simulink model "fopid"  (R2025b)
settings: Solver=FixedStepAuto  StartTime=0.0  StopTime=10.0  FixedStep=0.001  RelTol=1e-3
libraries: fod x1, slpidlib x1
settings Model: Creator=chen'z'y  LastModifiedBy=chen'z'y

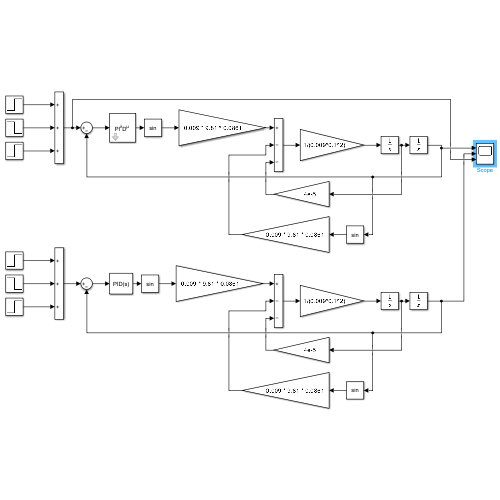
[thumbnail: Simulink's stored preview of the top-level diagram]
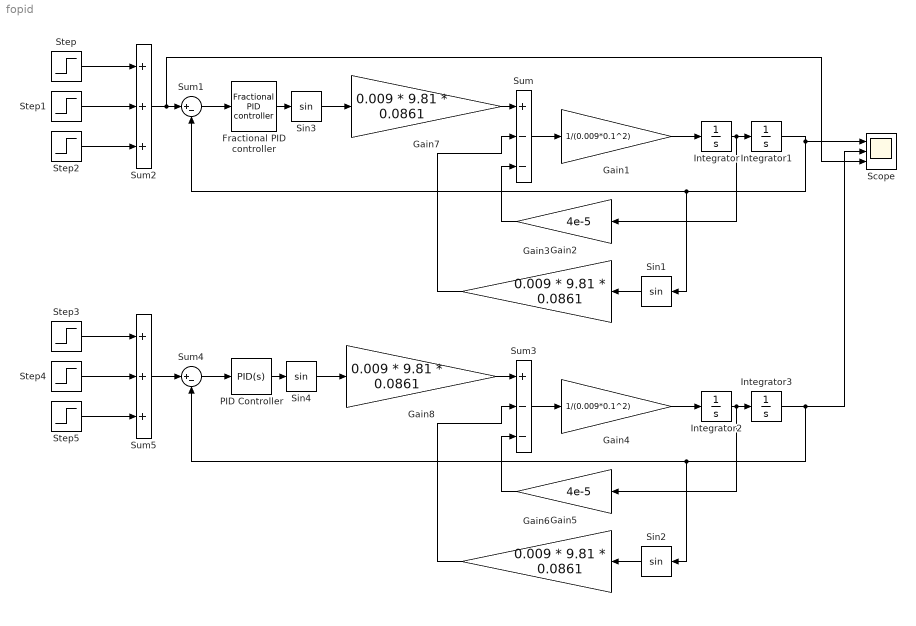
== system fopid ==
  Fractional PID controller : fod/Fractional PID controller  Kp=1  Ki=9.0747  lambda=0.95  Kd=0.3036  mic=0.95  freqRange=[0.01, 1000]  N=5
      settings: SourceProductName=FOMCON Toolbox
  Gain1 : Gain  Gain=1/(0.009*0.1^2)
  Gain2 : Gain  Gain=4e-5
  Gain{3,6..8} (4 alike) : Gain  Gain=0.009 * 9.81 * 0.0861
  Gain4 : Gain  Gain=1/(0.009*0.1^2)
  Gain5 : Gain  Gain=4e-5
  Integrator{,1..3} (4 alike) : Integrator
  PID Controller : slpidlib/PID Controller  Controller=PID  Form=Parallel  TimeDomain=Continuous-time  UseExternalTs=off  SampleTime=-1  IntegratorMethod=Forward Euler  FilterMethod=Forward Euler  ControllerParametersSource=internal  P=1  I=9.0747  UseKiTs=off  D=0.3036  UseExternalDerivativeSource=off  N=100  UseFilter=on  TunerSelectOption=Transfer Function Based (PID Tuner App)  InitialConditionSource=internal  InitialConditionForIntegrator=0  InitialConditionForFilter=0  DifferentiatorICPrevScaledInput=0  ExternalReset=none  TrackingMode=off  Kt=1  LimitOutput=off  SatLimitsSource=internal  UpperSaturationLimit=inf  LowerSaturationLimit=-inf  LinearizeAsGain=on  AntiWindupMode=none  Kb=1  LimitIntegrator=off  UpperIntegratorSaturationLimit=inf  LowerIntegratorSaturationLimit=-inf  POutMin=[]  POutMax=[]  IOutMin=[]  IOutMax=[]  DOutMin=[]  DOutMax=[]  NOutMin=[]  NOutMax=[]  SumOutMin=[]  SumOutMax=[]  SaturationOutMin=[]  SaturationOutMax=[]  PParamMin=[]  PParamMax=[]  IParamMin=[]  IParamMax=[]  DParamMin=[]  DParamMax=[]  NParamMin=[]  NParamMax=[]  KbParamMin=[]  KbParamMax=[]  KtParamMin=[]  KtParamMax=[]  KbOutMin=[]  KbOutMax=[]  KtOutMin=[]  KtOutMax=[]  IntegratorOutMin=[]  IntegratorOutMax=[]  FilterOutMin=[]  FilterOutMax=[]  SumI1OutMin=[]  SumI1OutMax=[]  SumI2OutMin=[]  SumI2OutMax=[]  SumI3OutMin=[]  SumI3OutMax=[]  SumI4OutMin=[]  SumI4OutMax=[]  SumDOutMin=[]  SumDOutMax=[]  DifferentiatorOutMin=[]  DifferentiatorOutMax=[]  FilterDiffOutCoefMin=[]  FilterDiffOutCoefMax=[]  ReciprocalOutMin=[]  ReciprocalOutMax=[]  SumDenOutMin=[]  SumDenOutMax=[]  SumNumOutMin=[]  SumNumOutMax=[]  DivideOutMin=[]  DivideOutMax=[]  UdiffTsProdOutMin=[]  UdiffTsProdOutMax=[]  NTsProdOutMin=[]  NTsProdOutMax=[]  UintegralTsProdOutMin=[]  UintegralTsProdOutMax=[]  UngainTsProdOutMin=[]  UngainTsProdOutMax=[]  ClampingZeroOutDataTypeStr=Inherit: Inherit via back propagation  ClampingZeroOutMin=[]  ClampingZeroOutMax=[]  FilterDenConstantOutDataTypeStr=Inherit: Inherit via back propagation  FilterDenConstantOutMin=[]  FilterDenConstantOutMax=[]  PCopyOutDataTypeStr=Inherit: Inherit via back propagation  PCopyOutMin=[]  PCopyOutMax=[]  NCopyOutDataTypeStr=Inherit: Inherit via back propagation  NCopyOutMin=[]  NCopyOutMax=[]  IntegratorContinuousStateAttributes=''  IntegratorStateMustResolveToSignalObject=off  IntegratorRTWStateStorageClass=Auto  FilterContinuousStateAttributes=''  FilterStateMustResolveToSignalObject=off  FilterRTWStateStorageClass=Auto  ParallelPVariant=InternalParameters  IdealPVariant=Disabled  IVariant=InternalParameters  DVariant=InternalParameters  IntegratorVariant=Continuous  SatVariant=Disabled  AWVariant=Passthrough  PCopyVariant=Disabled  TRVariant=Disabled  FdbkBlocksVariant=Forward  IdealPFdbkVariant=Disabled  SatFdbkVariant=Disabled  DerivativeFilterVariant=ContFilter  NVariant=InternalParameters  NCopyVariant=Disabled  FilterICVariant=InternalICsFilter  IntegratorICVariant=InternalICs  ExternalResetVariant=Disabled  TRSumVariant=Passthrough  SumFdbkVariant=Disabled  SumVariant=Sum_PID  TsampFilterVariant=InternalTs  TsampNgainVariant=Passthrough  TsampIntegralVariant=Disabled_SignalSpec  ExternalSaturationOutDataTypeStr=Inherit: Same as second input  DerivativeSourceVariant=ErrorSignal  PreIntVariant=InternalPreInt
  Scope : Scope  NumInputPorts=3
      settings: ActiveDisplayYMinimum=-0.1114400618964623  ActiveDisplayYMaximum=0.97065217865255393  DataLoggingVariableName=scope_data
  Sin{1..4} (4 alike) : Trigonometry
  Step : Step  Time=0  After=0.6  SampleTime=0
  Step1 : Step  Time=3  After=-0.35  SampleTime=0
  Step2 : Step  Time=7  After=0.5  SampleTime=0
  Step3 : Step  Time=0  After=0.6  SampleTime=0
  Step4 : Step  Time=3  After=-0.35  SampleTime=0
  Step5 : Step  Time=7  After=0.5  SampleTime=0
  Sum : Sum  Inputs=+--
  Sum1 : Sum  Inputs=|+-
  Sum2 : Sum  Inputs=+++
  Sum3 : Sum  Inputs=+--
  Sum4 : Sum  Inputs=|+-
  Sum5 : Sum  Inputs=+++
  wires:
  Sum/1 -> Gain1/1
  Gain1/1 -> Integrator/1
  Integrator/1 -> Gain2/1, Integrator1/1
  Sin1/1 -> Gain3/1
  Gain2/1 -> Sum/3
  Gain3/1 -> Sum/2
  Sum1/1 -> Fractional PID controller/1
  Integrator1/1 -> Scope/1, Sum1/2, Sin1/1
  Sum2/1 -> Scope/3, Sum1/1
  Step2/1 -> Sum2/3
  Step1/1 -> Sum2/2
  Step/1 -> Sum2/1
  Sum5/1 -> Sum4/1
  Gain5/1 -> Sum3/3
  Gain4/1 -> Integrator2/1
  Integrator3/1 -> Scope/2, Sin2/1, Sum4/2
  Sum3/1 -> Gain4/1
  Step5/1 -> Sum5/3
  Sin2/1 -> Gain6/1
  Step3/1 -> Sum5/1
  Gain6/1 -> Sum3/2
  Step4/1 -> Sum5/2
  Sum4/1 -> PID Controller/1
  Integrator2/1 -> Gain5/1, Integrator3/1
  Sin3/1 -> Gain7/1
  Gain7/1 -> Sum/1
  Fractional PID controller/1 -> Sin3/1
  Sin4/1 -> Gain8/1
  PID Controller/1 -> Sin4/1
  Gain8/1 -> Sum3/1
